simulink library "WECSim_Lib_Constraints"  (R2020b)
settings: Solver=VariableStepAuto  StartTime=0.0  StopTime=10.0  RelTol=1e-3
undefined symbols (not defined in the file or in its folder): constraint, simu, X, Y, Z
libraries: nesl_utility x48, sm_lib x34, WECSim_Lib_Body_Elements x1
(part 2 of 2)

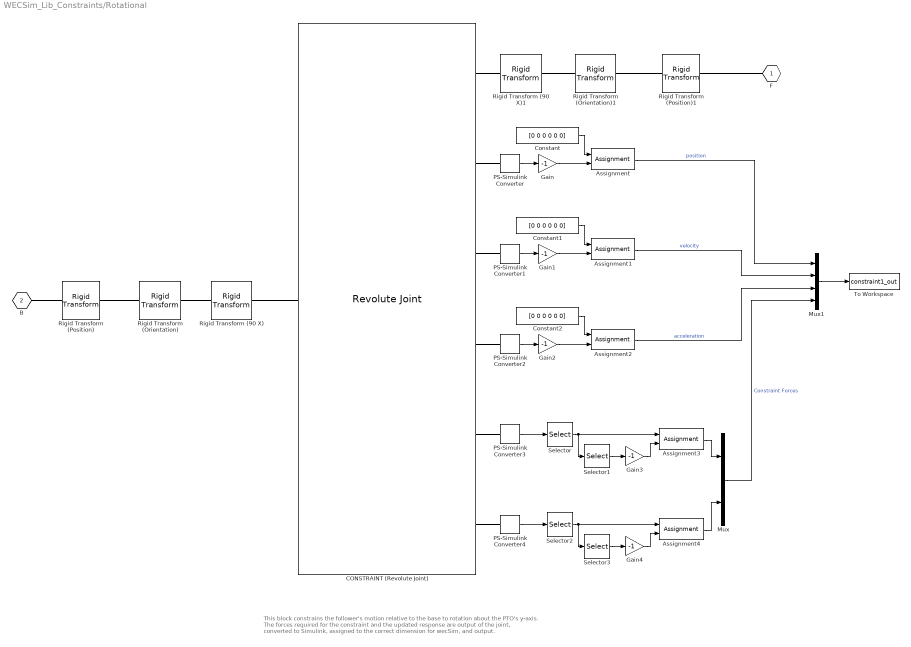
== system WECSim_Lib_Constraints/Rotational ==
  note: This block constrains the follower's motion relative to the base to rotation about the PTO's y-axis. The forces required for the constraint and the updated response are output of the joint, converted to Simulink, assigned to the correct dimension for wecSim, and output.
  Assignment : Assignment  DiagnosticForDimensions=Warning  IndexOptions=Index vector (dialog)  Indices=5  OutputSizes=1
  Assignment1 : Assignment  DiagnosticForDimensions=Warning  IndexOptions=Index vector (dialog)  Indices=5  OutputSizes=1
  Assignment2 : Assignment  DiagnosticForDimensions=Warning  IndexOptions=Index vector (dialog)  Indices=5  OutputSizes=1
  Assignment3 : Assignment  DiagnosticForDimensions=Warning  IndexOptions=Index vector (dialog)  Indices=2  OutputSizes=1
  Assignment4 : Assignment  DiagnosticForDimensions=Warning  IndexOptions=Index vector (dialog)  Indices=2  OutputSizes=1
  CONSTRAINT (Revolute Joint) : sm_lib/Joints/Revolute Joint  JointMode=Normal  CompositeWrenchDir=BaseOnFollower  CompositeWrenchFrame=BaseFrame  SenseConstraintForce=on  SenseConstraintTorque=on  SenseTotalForce=off  SenseTotalTorque=off  PositionTargetSpecify=off  PositionTargetPriority=High  PositionTargetValue=-constraint.extension.PositionTargetValue  PositionTargetValueUnits=deg  VelocityTargetSpecify=off  VelocityTargetPriority=High  VelocityTargetValue=0  VelocityTargetValueUnits=deg/s  EquilibriumPosition=0  EquilibriumPositionUnits=deg  SpringStiffness=0  SpringStiffnessUnits=N*m/deg  DampingCoefficient=0  DampingCoefficientUnits=N*m/(rad/s)  LowerLimitSpecify=off  LowerLimitBound=constraint.hardStops.lowerLimitBound  LowerLimitBoundUnits=deg  LowerLimitStiffness=constraint.hardStops.lowerLimitStiffness  LowerLimitStiffnessUnits=N*m/deg  LowerLimitDamping=constraint.hardStops.lowerLimitDamping  LowerLimitDampingUnits=N*m/(deg/s)  LowerLimitTransitionRegionWidth=constraint.hardStops.lowerLimitTransitionRegionWidth  LowerLimitTransitionRegionWidthUnits=deg  UpperLimitSpecify=off  UpperLimitBound=constraint.hardStops.upperLimitBound  UpperLimitBoundUnits=deg  UpperLimitStiffness=constraint.hardStops.upperLimitStiffness  UpperLimitStiffnessUnits=N*m/deg  UpperLimitDamping=constraint.hardStops.upperLimitDamping  UpperLimitDampingUnits=N*m/(deg/s)  UpperLimitTransitionRegionWidth=constraint.hardStops.upperLimitTransitionRegionWidth  UpperLimitTransitionRegionWidthUnits=deg  TorqueActuationMode=NoTorque  MotionActuationMode=ComputedMotion  SensePosition=on  SenseVelocity=on  SenseAcceleration=on  SenseTorqueForce=off  SenseLowerLimitTorqueForce=off  SenseUpperLimitTorqueForce=off
  Constant : Constant  Value=[0 0 0 0 0 0]
  Constant1 : Constant  Value=[0 0 0 0 0 0]
  Constant2 : Constant  Value=[0 0 0 0 0 0]
  Gain{,1..4} (5 alike) : Gain  Gain=-1
  Mux : Mux  Inputs=2
  Mux1 : Mux
  PS-Simulink Converter{,1..4} (5 alike) : nesl_utility/PS-Simulink Converter  PhysicalDomain=network_engine_domain  SubClassName=ps_output  LeftPortType=input  RightPortType=output  PseudoPeriodic=off  Frequencies=[]  VectorFormat=1-D array  Unit=1  AffineConversion=off
  Rigid Transform (Position) : sm_lib/Frames and Transforms/Rigid Transform  RotationMethod=None  FollAlignAxisA=+X  BaseAlignAxisA=+Y  FollAlignAxisB=+Y  BaseAlignAxisB=+Z  RotationStandardAxis=+Y  RotationAngle=0  RotationAngleUnits=rad  RotationArbitraryAxis=[0 1 0]  RotationSequenceAxes=FollowerAxes  RotationSequence=XYX  RotationSequenceAngles=[0 0 0]  RotationSequenceAnglesUnits=deg  RotationMatrix=[1 0 0; 0 1 0; 0 0 1]  Quaternion=[1 0 0 0]  TranslationMethod=Cartesian  TranslationCartesianOffset=constraint.initial.displacement+constraint.location  TranslationCartesianOffsetUnits=m  TranslationStandardAxis=+Z  TranslationStandardOffset=0  TranslationStandardOffsetUnits=m  TranslationROffset=0  TranslationROffsetUnits=m  TranslationThetaOffset=0  TranslationThetaOffsetUnits=deg  TranslationZOffset=0  TranslationZOffsetUnits=m
  Rigid Transform (Position)1 : sm_lib/Frames and Transforms/Rigid Transform  RotationMethod=None  FollAlignAxisA=+X  BaseAlignAxisA=+Y  FollAlignAxisB=+Y  BaseAlignAxisB=+Z  RotationStandardAxis=+Y  RotationAngle=0  RotationAngleUnits=rad  RotationArbitraryAxis=[0 1 0]  RotationSequenceAxes=FollowerAxes  RotationSequence=XYX  RotationSequenceAngles=[0 0 0]  RotationSequenceAnglesUnits=deg  RotationMatrix=[1 0 0; 0 1 0; 0 0 1]  Quaternion=[1 0 0 0]  TranslationMethod=Cartesian  TranslationCartesianOffset=constraint.initial.displacement+constraint.location  TranslationCartesianOffsetUnits=m  TranslationStandardAxis=+Z  TranslationStandardOffset=0  TranslationStandardOffsetUnits=m  TranslationROffset=0  TranslationROffsetUnits=m  TranslationThetaOffset=0  TranslationThetaOffsetUnits=deg  TranslationZOffset=0  TranslationZOffsetUnits=m
  Rigid Transform (90 X) : sm_lib/Frames and Transforms/Rigid Transform  RotationMethod=StandardAxis  FollAlignAxisA=+X  BaseAlignAxisA=+Y  FollAlignAxisB=+Y  BaseAlignAxisB=+Z  RotationStandardAxis=+X  RotationAngle=90  RotationAngleUnits=deg  RotationArbitraryAxis=[0 1 0]  RotationSequenceAxes=FollowerAxes  RotationSequence=XYX  RotationSequenceAngles=[0 0 0]  RotationSequenceAnglesUnits=deg  RotationMatrix=[1 0 0; 0 1 0; 0 0 1]  Quaternion=[1 0 0 0]  TranslationMethod=None  TranslationCartesianOffset=constraint.location  TranslationCartesianOffsetUnits=m  TranslationStandardAxis=+Z  TranslationStandardOffset=0  TranslationStandardOffsetUnits=m  TranslationROffset=0  TranslationROffsetUnits=m  TranslationThetaOffset=0  TranslationThetaOffsetUnits=deg  TranslationZOffset=0  TranslationZOffsetUnits=m
  Rigid Transform (90 X)1 : sm_lib/Frames and Transforms/Rigid Transform  RotationMethod=StandardAxis  FollAlignAxisA=+X  BaseAlignAxisA=+Y  FollAlignAxisB=+Y  BaseAlignAxisB=+Z  RotationStandardAxis=+X  RotationAngle=90  RotationAngleUnits=deg  RotationArbitraryAxis=[0 1 0]  RotationSequenceAxes=FollowerAxes  RotationSequence=XYX  RotationSequenceAngles=[0 0 0]  RotationSequenceAnglesUnits=deg  RotationMatrix=[1 0 0; 0 1 0; 0 0 1]  Quaternion=[1 0 0 0]  TranslationMethod=None  TranslationCartesianOffset=constraint.location  TranslationCartesianOffsetUnits=m  TranslationStandardAxis=+Z  TranslationStandardOffset=0  TranslationStandardOffsetUnits=m  TranslationROffset=0  TranslationROffsetUnits=m  TranslationThetaOffset=0  TranslationThetaOffsetUnits=deg  TranslationZOffset=0  TranslationZOffsetUnits=m
  Rigid Transform (Orientation) : sm_lib/Frames and Transforms/Rigid Transform  RotationMethod=RotationMatrix  FollAlignAxisA=+X  BaseAlignAxisA=+Y  FollAlignAxisB=+Y  BaseAlignAxisB=+Z  RotationStandardAxis=+Y  RotationAngle=0  RotationAngleUnits=rad  RotationArbitraryAxis=[0 1 0]  RotationSequenceAxes=FollowerAxes  RotationSequence=XYX  RotationSequenceAngles=[0 0 0]  RotationSequenceAnglesUnits=deg  RotationMatrix=constraint.orientation.rotationMatrix  Quaternion=[1 0 0 0]  TranslationMethod=None  TranslationCartesianOffset=constraint.location  TranslationCartesianOffsetUnits=m  TranslationStandardAxis=+Z  TranslationStandardOffset=0  TranslationStandardOffsetUnits=m  TranslationROffset=0  TranslationROffsetUnits=m  TranslationThetaOffset=0  TranslationThetaOffsetUnits=deg  TranslationZOffset=0  TranslationZOffsetUnits=m
  Rigid Transform (Orientation)1 : sm_lib/Frames and Transforms/Rigid Transform  RotationMethod=RotationMatrix  FollAlignAxisA=+X  BaseAlignAxisA=+Y  FollAlignAxisB=+Y  BaseAlignAxisB=+Z  RotationStandardAxis=+Y  RotationAngle=0  RotationAngleUnits=rad  RotationArbitraryAxis=[0 1 0]  RotationSequenceAxes=FollowerAxes  RotationSequence=XYX  RotationSequenceAngles=[0 0 0]  RotationSequenceAnglesUnits=deg  RotationMatrix=constraint.orientation.rotationMatrix  Quaternion=[1 0 0 0]  TranslationMethod=None  TranslationCartesianOffset=constraint.location  TranslationCartesianOffsetUnits=m  TranslationStandardAxis=+Z  TranslationStandardOffset=0  TranslationStandardOffsetUnits=m  TranslationROffset=0  TranslationROffsetUnits=m  TranslationThetaOffset=0  TranslationThetaOffsetUnits=deg  TranslationZOffset=0  TranslationZOffsetUnits=m
  Selector : Selector  InputPortWidth=3  IndexOptions=Index vector (dialog)  Indices=[1 3 2]  OutputSizes=1
  Selector1 : Selector  InputPortWidth=3  IndexOptions=Index vector (dialog)  Indices=[2]  OutputSizes=1
  Selector2 : Selector  InputPortWidth=3  IndexOptions=Index vector (dialog)  Indices=[1 3 2]  OutputSizes=1
  Selector3 : Selector  InputPortWidth=3  IndexOptions=Index vector (dialog)  Indices=[2]  OutputSizes=1
  To Workspace : ToWorkspace  VariableName=constraint1_out  SaveFormat=Structure With Time  SampleTime=simu.dtOut
  F : PMIOPort  Side=Right
  B : PMIOPort  Port=2  Side=Left
  wires:
  Assignment4/1 -> Mux/2
  PS-Simulink Converter4/1 -> Selector2/1
  Gain4/1 -> Assignment4/2
  Selector3/1 -> Gain4/1
  Selector2/1 -> Assignment4/1, Selector3/1
  Assignment3/1 -> Mux/1
  Gain3/1 -> Assignment3/2
  Selector1/1 -> Gain3/1
  Selector/1 -> Selector1/1, Assignment3/1
  PS-Simulink Converter3/1 -> Selector/1
  Gain2/1 -> Assignment2/2
  Gain1/1 -> Assignment1/2
  Gain/1 -> Assignment/2
  Constant/1 -> Assignment/1
  Constant1/1 -> Assignment1/1
  Constant2/1 -> Assignment2/1
  Assignment2/1 -> Mux1/3  "acceleration"
  Assignment1/1 -> Mux1/2  "velocity"
  Assignment/1 -> Mux1/1  "position"
  Mux/1 -> Mux1/4  "Constraint Forces"
  Mux1/1 -> To Workspace/1
  PS-Simulink Converter/1 -> Gain/1
  PS-Simulink Converter1/1 -> Gain1/1
  PS-Simulink Converter2/1 -> Gain2/1
  connections:
  Rigid Transform (Position)1/LConn1 -- F/RConn1
  Rigid Transform (Position)1/RConn1 -- Rigid Transform (Orientation)1/LConn1
  Rigid Transform (90 X)1/RConn1 -- CONSTRAINT (Revolute Joint)/RConn1
  Rigid Transform (Orientation)1/RConn1 -- Rigid Transform (90 X)1/LConn1
  Rigid Transform (90 X)/RConn1 -- CONSTRAINT (Revolute Joint)/LConn1
  Rigid Transform (Orientation)/RConn1 -- Rigid Transform (90 X)/LConn1
  Rigid Transform (Position)/RConn1 -- Rigid Transform (Orientation)/LConn1
  Rigid Transform (Position)/LConn1 -- B/RConn1
  CONSTRAINT (Revolute Joint)/RConn4 -- PS-Simulink Converter2/LConn1
  CONSTRAINT (Revolute Joint)/RConn3 -- PS-Simulink Converter1/LConn1
  CONSTRAINT (Revolute Joint)/RConn2 -- PS-Simulink Converter/LConn1
  PS-Simulink Converter4/LConn1 -- CONSTRAINT (Revolute Joint)/RConn6
  PS-Simulink Converter3/LConn1 -- CONSTRAINT (Revolute Joint)/RConn5

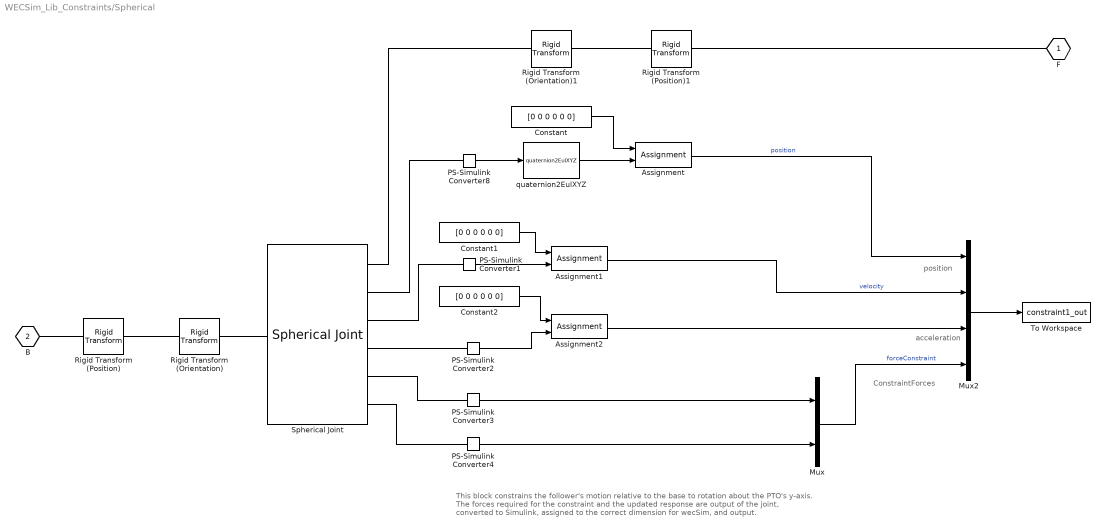
== system WECSim_Lib_Constraints/Spherical ==
  note: This block constrains the follower's motion relative to the base to rotation about the PTO's y-axis. The forces required for the constraint and the updated response are output of the joint, converted to Simulink, assigned to the correct dimension for wecSim, and output.
  note: acceleration
  note: ConstraintForces
  note: position
  "Assignment " : Assignment  IndexOptions=Index vector (dialog)  Indices=[4 5 6]  OutputSizes=1
  Assignment1 : Assignment  IndexOptions=Index vector (dialog)  Indices=[4 5 6]  OutputSizes=1
  Assignment2 : Assignment  IndexOptions=Index vector (dialog)  Indices=[4,5,6]  OutputSizes=1
  Constant : Constant  Value=[0 0 0 0 0 0]
  Constant1 : Constant  Value=[0 0 0 0 0 0]
  Constant2 : Constant  Value=[0 0 0 0 0 0]
  Mux : Mux  Inputs=2
  Mux2 : Mux
  PS-Simulink Converter{1..4,8} (5 alike) : nesl_utility/PS-Simulink Converter  PhysicalDomain=network_engine_domain  SubClassName=ps_output  LeftPortType=input  RightPortType=output  PseudoPeriodic=off  Frequencies=[]  VectorFormat=1-D array  Unit=inherit  AffineConversion=off
  Rigid Transform (Orientation) : sm_lib/Frames and Transforms/Rigid Transform  RotationMethod=RotationMatrix  FollAlignAxisA=+X  BaseAlignAxisA=+Y  FollAlignAxisB=+Y  BaseAlignAxisB=+Z  RotationStandardAxis=+Z  RotationAngle=0.0  RotationAngleUnits=deg  RotationArbitraryAxis=[0 0 1]  RotationSequenceAxes=FollowerAxes  RotationSequence=XYX  RotationSequenceAngles=[0 0 0]  RotationSequenceAnglesUnits=deg  RotationMatrix=constraint.orientation.rotationMatrix  Quaternion=[1 0 0 0]  TranslationMethod=None  TranslationCartesianOffset=constraint.initial.displacement+constraint.location  TranslationCartesianOffsetUnits=m  TranslationStandardAxis=+Z  TranslationStandardOffset=0  TranslationStandardOffsetUnits=m  TranslationROffset=0  TranslationROffsetUnits=m  TranslationThetaOffset=0  TranslationThetaOffsetUnits=deg  TranslationZOffset=0  TranslationZOffsetUnits=m
  Rigid Transform (Orientation)1 : sm_lib/Frames and Transforms/Rigid Transform  RotationMethod=RotationMatrix  FollAlignAxisA=+X  BaseAlignAxisA=+Y  FollAlignAxisB=+Y  BaseAlignAxisB=+Z  RotationStandardAxis=+Z  RotationAngle=0.0  RotationAngleUnits=deg  RotationArbitraryAxis=[0 0 1]  RotationSequenceAxes=FollowerAxes  RotationSequence=XYX  RotationSequenceAngles=[0 0 0]  RotationSequenceAnglesUnits=deg  RotationMatrix=constraint.orientation.rotationMatrix  Quaternion=[1 0 0 0]  TranslationMethod=None  TranslationCartesianOffset=constraint.initial.displacement+constraint.location  TranslationCartesianOffsetUnits=m  TranslationStandardAxis=+Z  TranslationStandardOffset=0  TranslationStandardOffsetUnits=m  TranslationROffset=0  TranslationROffsetUnits=m  TranslationThetaOffset=0  TranslationThetaOffsetUnits=deg  TranslationZOffset=0  TranslationZOffsetUnits=m
  Rigid Transform (Position) : sm_lib/Frames and Transforms/Rigid Transform  RotationMethod=None  FollAlignAxisA=+X  BaseAlignAxisA=+Y  FollAlignAxisB=+Y  BaseAlignAxisB=+Z  RotationStandardAxis=+Z  RotationAngle=0.0  RotationAngleUnits=deg  RotationArbitraryAxis=[0 0 1]  RotationSequenceAxes=FollowerAxes  RotationSequence=XYX  RotationSequenceAngles=[0 0 0]  RotationSequenceAnglesUnits=deg  RotationMatrix=[1 0 0; 0 1 0; 0 0 1]  Quaternion=[1 0 0 0]  TranslationMethod=Cartesian  TranslationCartesianOffset=constraint.initial.displacement+constraint.location  TranslationCartesianOffsetUnits=m  TranslationStandardAxis=+Z  TranslationStandardOffset=0  TranslationStandardOffsetUnits=m  TranslationROffset=0  TranslationROffsetUnits=m  TranslationThetaOffset=0  TranslationThetaOffsetUnits=deg  TranslationZOffset=0  TranslationZOffsetUnits=m
  Rigid Transform (Position)1 : sm_lib/Frames and Transforms/Rigid Transform  RotationMethod=None  FollAlignAxisA=+X  BaseAlignAxisA=+Y  FollAlignAxisB=+Y  BaseAlignAxisB=+Z  RotationStandardAxis=+Z  RotationAngle=0.0  RotationAngleUnits=deg  RotationArbitraryAxis=[0 0 1]  RotationSequenceAxes=FollowerAxes  RotationSequence=XYX  RotationSequenceAngles=[0 0 0]  RotationSequenceAnglesUnits=deg  RotationMatrix=[1 0 0; 0 1 0; 0 0 1]  Quaternion=[1 0 0 0]  TranslationMethod=Cartesian  TranslationCartesianOffset=constraint.initial.displacement+constraint.location  TranslationCartesianOffsetUnits=m  TranslationStandardAxis=+Z  TranslationStandardOffset=0  TranslationStandardOffsetUnits=m  TranslationROffset=0  TranslationROffsetUnits=m  TranslationThetaOffset=0  TranslationThetaOffsetUnits=deg  TranslationZOffset=0  TranslationZOffsetUnits=m
  Spherical Joint : sm_lib/Joints/Spherical Joint  JointMode=Normal  CompositeWrenchDir=BaseOnFollower  CompositeWrenchFrame=BaseFrame  SenseConstraintForce=on  SenseConstraintTorque=on  SenseTotalForce=off  SenseTotalTorque=off  PositionTargetSpecify=off  PositionTargetPriority=High  PositionTargetRotationMethod=RotationSequence  PositionTargetFollAlignAxisA=+X  PositionTargetBaseAlignAxisA=+Y  PositionTargetFollAlignAxisB=+Y  PositionTargetBaseAlignAxisB=+Z  PositionTargetRotationStandardAxis=+Z  PositionTargetRotationAngle=0.0  PositionTargetRotationAngleUnits=deg  PositionTargetRotationArbitraryAxis=[0 0 1]  PositionTargetRotationSequenceAxes=BaseAxes  PositionTargetRotationSequence=XYZ  PositionTargetRotationSequenceAngles=constraint.extension.PositionTargetValue  PositionTargetRotationSequenceAnglesUnits=deg  PositionTargetRotationMatrix=[1 0 0; 0 1 0; 0 0 1]  PositionTargetQuaternion=[1 0 0 0]  VelocityTargetSpecify=off  VelocityTargetPriority=High  VelocityTargetValue=[0 0 0]  VelocityTargetValueUnits=deg/s  VelocityTargetInFollowerFrame=on  EqPosRotationMethod=None  EqPosFollAlignAxisA=+X  EqPosBaseAlignAxisA=+Y  EqPosFollAlignAxisB=+Y  EqPosBaseAlignAxisB=+Z  EqPosRotationStandardAxis=+Z  EqPosRotationAngle=0.0  EqPosRotationAngleUnits=deg  EqPosRotationArbitraryAxis=[0 0 1]  EqPosRotationSequenceAxes=FollowerAxes  EqPosRotationSequence=XYX  EqPosRotationSequenceAngles=[0 0 0]  EqPosRotationSequenceAnglesUnits=deg  EqPosRotationMatrix=[1 0 0; 0 1 0; 0 0 1]  EqPosQuaternion=[1 0 0 0]  SpringStiffness=0  SpringStiffnessUnits=N*m/deg  DampingCoefficient=0  DampingCoefficientUnits=N*m/(deg/s)  LowerLimitSpecify=off  LowerLimitBound=15  LowerLimitBoundUnits=deg  LowerLimitStiffness=1e4  LowerLimitStiffnessUnits=N*m/deg  LowerLimitDamping=10  LowerLimitDampingUnits=N*m/(deg/s)  LowerLimitTransitionRegionWidth=0.1  LowerLimitTransitionRegionWidthUnits=deg  UpperLimitSpecify=off  UpperLimitBound=45  UpperLimitBoundUnits=deg  UpperLimitStiffness=1e4  UpperLimitStiffnessUnits=N*m/deg  UpperLimitDamping=10  UpperLimitDampingUnits=N*m/(deg/s)  UpperLimitTransitionRegionWidth=0.1  UpperLimitTransitionRegionWidthUnits=deg  TorqueActuationMode=NoTorque  ActuateTorqueX=off  ActuateTorqueY=off  ActuateTorqueZ=off  ActuateTorque=off  ActuationFrame=BaseFrame  SensePosition=on  SenseVelocityX=off  SenseVelocityY=off  SenseVelocityZ=off  SenseVelocity=on  SenseAccelerationX=off  SenseAccelerationY=off  SenseAccelerationZ=off  SenseAcceleration=on  SenseLowerLimitTorqueMag=off  SenseUpperLimitTorqueMag=off  SensingFrame=BaseFrame
  To Workspace : ToWorkspace  VariableName=constraint1_out  SaveFormat=Structure With Time  SampleTime=simu.dtOut
  quaternion2EulXYZ : WECSim_Lib_Body_Elements/Rigid Body/Hydrodynamic Body/Structure/Motion Sensor/quaternion2EulXYZ  SystemSampleTime=-1  VariantActivationTime=update diagram  Latency=0  AutoFrameSizeCalculation=off
  F : PMIOPort  Side=Right
  B : PMIOPort  Port=2  Side=Left
  wires:
  quaternion2EulXYZ/1 -> "Assignment "/2
  Constant2/1 -> Assignment2/1
  PS-Simulink Converter2/1 -> Assignment2/2
  PS-Simulink Converter1/1 -> Assignment1/2
  Mux2/1 -> To Workspace/1
  "Assignment "/1 -> Mux2/1  "position"
  Constant/1 -> "Assignment "/1
  Constant1/1 -> Assignment1/1
  Assignment1/1 -> Mux2/2  "velocity"
  PS-Simulink Converter4/1 -> Mux/2
  PS-Simulink Converter8/1 -> quaternion2EulXYZ/1
  Assignment2/1 -> Mux2/3
  PS-Simulink Converter3/1 -> Mux/1
  Mux/1 -> Mux2/4  "forceConstraint"
  connections:
  Spherical Joint/RConn2 -- PS-Simulink Converter8/LConn1
  Spherical Joint/RConn3 -- PS-Simulink Converter1/LConn1
  Rigid Transform (Position)1/LConn1 -- F/RConn1
  Rigid Transform (Orientation)/RConn1 -- Spherical Joint/LConn1
  Spherical Joint/RConn6 -- PS-Simulink Converter4/LConn1
  Rigid Transform (Position)/LConn1 -- B/RConn1
  Spherical Joint/RConn5 -- PS-Simulink Converter3/LConn1
  Rigid Transform (Orientation)/LConn1 -- Rigid Transform (Position)/RConn1
  Spherical Joint/RConn4 -- PS-Simulink Converter2/LConn1
  Rigid Transform (Orientation)1/LConn1 -- Rigid Transform (Position)1/RConn1
  Spherical Joint/RConn1 -- Rigid Transform (Orientation)1/RConn1

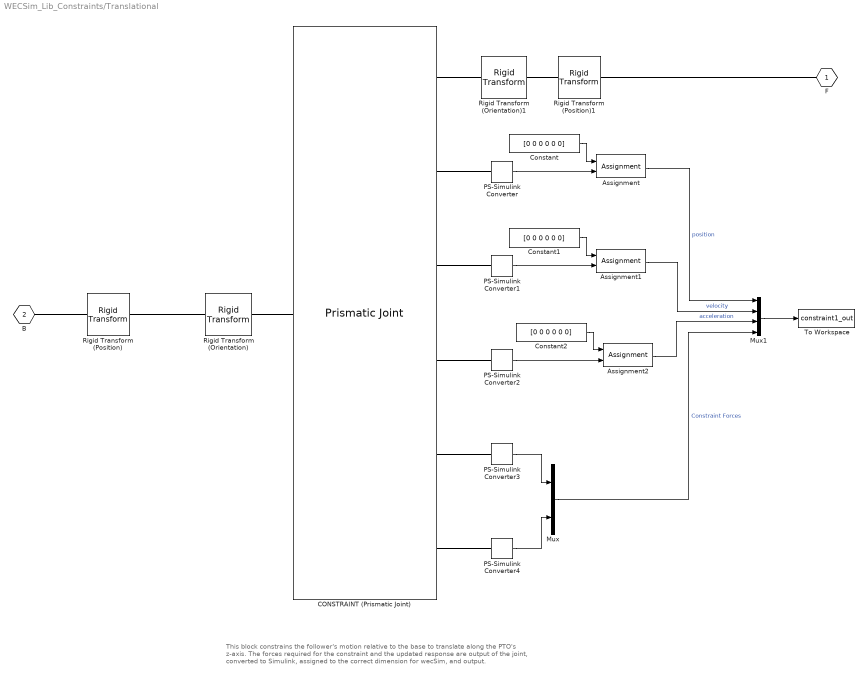
== system WECSim_Lib_Constraints/Translational ==
  note: This block constrains the follower's motion relative to the base to translate along the PTO's z-axis. The forces required for the constraint and the updated response are output of the joint, converted to Simulink, assigned to the correct dimension for wecSim, and output.
  Assignment : Assignment  DiagnosticForDimensions=Warning  IndexOptions=Index vector (dialog)  Indices=3  OutputSizes=1
  Assignment1 : Assignment  DiagnosticForDimensions=Warning  IndexOptions=Index vector (dialog)  Indices=3  OutputSizes=1
  Assignment2 : Assignment  DiagnosticForDimensions=Warning  IndexOptions=Index vector (dialog)  Indices=3  OutputSizes=1
  CONSTRAINT (Prismatic Joint) : sm_lib/Joints/Prismatic Joint  JointMode=Normal  CompositeWrenchDir=BaseOnFollower  CompositeWrenchFrame=BaseFrame  SenseConstraintForce=on  SenseConstraintTorque=on  SenseTotalForce=off  SenseTotalTorque=off  PositionTargetSpecify=off  PositionTargetPriority=High  PositionTargetValue=constraint.extension.PositionTargetValue  PositionTargetValueUnits=m  VelocityTargetSpecify=off  VelocityTargetPriority=High  VelocityTargetValue=0  VelocityTargetValueUnits=m/s  EquilibriumPosition=0  EquilibriumPositionUnits=m  SpringStiffness=0  SpringStiffnessUnits=N/m  DampingCoefficient=0  DampingCoefficientUnits=N/(m/s)  LowerLimitSpecify=off  LowerLimitBound=constraint.hardStops.lowerLimitBound  LowerLimitBoundUnits=m  LowerLimitStiffness=constraint.hardStops.lowerLimitStiffness  LowerLimitStiffnessUnits=N/m  LowerLimitDamping=constraint.hardStops.lowerLimitDamping  LowerLimitDampingUnits=N/(m/s)  LowerLimitTransitionRegionWidth=constraint.hardStops.lowerLimitTransitionRegionWidth  LowerLimitTransitionRegionWidthUnits=m  UpperLimitSpecify=off  UpperLimitBound=constraint.hardStops.upperLimitBound  UpperLimitBoundUnits=m  UpperLimitStiffness=constraint.hardStops.upperLimitStiffness  UpperLimitStiffnessUnits=N/m  UpperLimitDamping=constraint.hardStops.upperLimitDamping  UpperLimitDampingUnits=N/(m/s)  UpperLimitTransitionRegionWidth=constraint.hardStops.upperLimitTransitionRegionWidth  UpperLimitTransitionRegionWidthUnits=m  TorqueActuationMode=NoTorque  MotionActuationMode=ComputedMotion  SensePosition=on  SenseVelocity=on  SenseAcceleration=on  SenseTorqueForce=off  SenseLowerLimitTorqueForce=off  SenseUpperLimitTorqueForce=off
  Constant : Constant  Value=[0 0 0 0 0 0]
  Constant1 : Constant  Value=[0 0 0 0 0 0]
  Constant2 : Constant  Value=[0 0 0 0 0 0]
  Mux : Mux  Inputs=2
  Mux1 : Mux
  PS-Simulink Converter{,1..4} (5 alike) : nesl_utility/PS-Simulink Converter  PhysicalDomain=network_engine_domain  SubClassName=ps_output  LeftPortType=input  RightPortType=output  PseudoPeriodic=off  Frequencies=[]  VectorFormat=1-D array  Unit=1  AffineConversion=off
  Rigid Transform (Position) : sm_lib/Frames and Transforms/Rigid Transform  RotationMethod=None  FollAlignAxisA=+X  BaseAlignAxisA=+Y  FollAlignAxisB=+Y  BaseAlignAxisB=+Z  RotationStandardAxis=+Y  RotationAngle=0  RotationAngleUnits=rad  RotationArbitraryAxis=[0 1 0]  RotationSequenceAxes=FollowerAxes  RotationSequence=XYX  RotationSequenceAngles=[0 0 0]  RotationSequenceAnglesUnits=deg  RotationMatrix=[1 0 0; 0 1 0; 0 0 1]  Quaternion=[1 0 0 0]  TranslationMethod=Cartesian  TranslationCartesianOffset=constraint.initial.displacement+constraint.location  TranslationCartesianOffsetUnits=m  TranslationStandardAxis=+Z  TranslationStandardOffset=0  TranslationStandardOffsetUnits=m  TranslationROffset=0  TranslationROffsetUnits=m  TranslationThetaOffset=0  TranslationThetaOffsetUnits=deg  TranslationZOffset=0  TranslationZOffsetUnits=m
  Rigid Transform (Position)1 : sm_lib/Frames and Transforms/Rigid Transform  RotationMethod=None  FollAlignAxisA=+X  BaseAlignAxisA=+Y  FollAlignAxisB=+Y  BaseAlignAxisB=+Z  RotationStandardAxis=+Y  RotationAngle=0  RotationAngleUnits=rad  RotationArbitraryAxis=[0 1 0]  RotationSequenceAxes=FollowerAxes  RotationSequence=XYX  RotationSequenceAngles=[0 0 0]  RotationSequenceAnglesUnits=deg  RotationMatrix=[1 0 0; 0 1 0; 0 0 1]  Quaternion=[1 0 0 0]  TranslationMethod=Cartesian  TranslationCartesianOffset=constraint.initial.displacement+constraint.location  TranslationCartesianOffsetUnits=m  TranslationStandardAxis=+Z  TranslationStandardOffset=0  TranslationStandardOffsetUnits=m  TranslationROffset=0  TranslationROffsetUnits=m  TranslationThetaOffset=0  TranslationThetaOffsetUnits=deg  TranslationZOffset=0  TranslationZOffsetUnits=m
  Rigid Transform (Orientation) : sm_lib/Frames and Transforms/Rigid Transform  RotationMethod=RotationMatrix  FollAlignAxisA=+X  BaseAlignAxisA=+Y  FollAlignAxisB=+Y  BaseAlignAxisB=+Z  RotationStandardAxis=+Y  RotationAngle=0  RotationAngleUnits=rad  RotationArbitraryAxis=[0 1 0]  RotationSequenceAxes=FollowerAxes  RotationSequence=XYX  RotationSequenceAngles=[0 0 0]  RotationSequenceAnglesUnits=deg  RotationMatrix=constraint.orientation.rotationMatrix  Quaternion=[1 0 0 0]  TranslationMethod=None  TranslationCartesianOffset=constraint.location  TranslationCartesianOffsetUnits=m  TranslationStandardAxis=+Z  TranslationStandardOffset=0  TranslationStandardOffsetUnits=m  TranslationROffset=0  TranslationROffsetUnits=m  TranslationThetaOffset=0  TranslationThetaOffsetUnits=deg  TranslationZOffset=0  TranslationZOffsetUnits=m
  Rigid Transform (Orientation)1 : sm_lib/Frames and Transforms/Rigid Transform  RotationMethod=RotationMatrix  FollAlignAxisA=+X  BaseAlignAxisA=+Y  FollAlignAxisB=+Y  BaseAlignAxisB=+Z  RotationStandardAxis=+Y  RotationAngle=0  RotationAngleUnits=rad  RotationArbitraryAxis=[0 1 0]  RotationSequenceAxes=FollowerAxes  RotationSequence=XYX  RotationSequenceAngles=[0 0 0]  RotationSequenceAnglesUnits=deg  RotationMatrix=constraint.orientation.rotationMatrix  Quaternion=[1 0 0 0]  TranslationMethod=None  TranslationCartesianOffset=constraint.location  TranslationCartesianOffsetUnits=m  TranslationStandardAxis=+Z  TranslationStandardOffset=0  TranslationStandardOffsetUnits=m  TranslationROffset=0  TranslationROffsetUnits=m  TranslationThetaOffset=0  TranslationThetaOffsetUnits=deg  TranslationZOffset=0  TranslationZOffsetUnits=m
  To Workspace : ToWorkspace  VariableName=constraint1_out  SaveFormat=Structure With Time  SampleTime=simu.dtOut
  F : PMIOPort  Side=Right
  B : PMIOPort  Port=2  Side=Left
  wires:
  Constant2/1 -> Assignment2/1
  PS-Simulink Converter2/1 -> Assignment2/2
  Constant1/1 -> Assignment1/1
  PS-Simulink Converter1/1 -> Assignment1/2
  Constant/1 -> Assignment/1
  Assignment/1 -> Mux1/1  "position"
  PS-Simulink Converter4/1 -> Mux/2
  PS-Simulink Converter3/1 -> Mux/1
  Mux/1 -> Mux1/4  "Constraint Forces"
  Assignment2/1 -> Mux1/3  "acceleration"
  Assignment1/1 -> Mux1/2  "velocity"
  PS-Simulink Converter/1 -> Assignment/2
  Mux1/1 -> To Workspace/1
  connections:
  Rigid Transform (Position)1/RConn1 -- Rigid Transform (Orientation)1/LConn1
  Rigid Transform (Orientation)/RConn1 -- CONSTRAINT (Prismatic Joint)/LConn1
  Rigid Transform (Position)/RConn1 -- Rigid Transform (Orientation)/LConn1
  Rigid Transform (Position)/LConn1 -- B/RConn1
  Rigid Transform (Orientation)1/RConn1 -- CONSTRAINT (Prismatic Joint)/RConn1
  CONSTRAINT (Prismatic Joint)/RConn4 -- PS-Simulink Converter2/LConn1
  CONSTRAINT (Prismatic Joint)/RConn3 -- PS-Simulink Converter1/LConn1
  PS-Simulink Converter/LConn1 -- CONSTRAINT (Prismatic Joint)/RConn2
  PS-Simulink Converter4/LConn1 -- CONSTRAINT (Prismatic Joint)/RConn6
  PS-Simulink Converter3/LConn1 -- CONSTRAINT (Prismatic Joint)/RConn5
  Rigid Transform (Position)1/LConn1 -- F/RConn1
